simulink model "ZF02HD250606_23a"  (R2023a)
settings: Solver=ode4  StartTime=0.0  StopTime=inf  FixedStep=0.002  RelTol=1e-3
InitFcn:
  |  T_c = 0.002;
undefined symbols (not defined in the file): DiscIntNeverNeededParam, Discrete, magnitude, Time
libraries: AFCToolbox x33, simulink x28, simulink_extras x7, sharedtransform x2, ctrlSharedLib x2, aerolibconvert2 x1, aerolibtransform2 x1, dspstat3 x1, dspsolvers x1
(part 2 of 3)

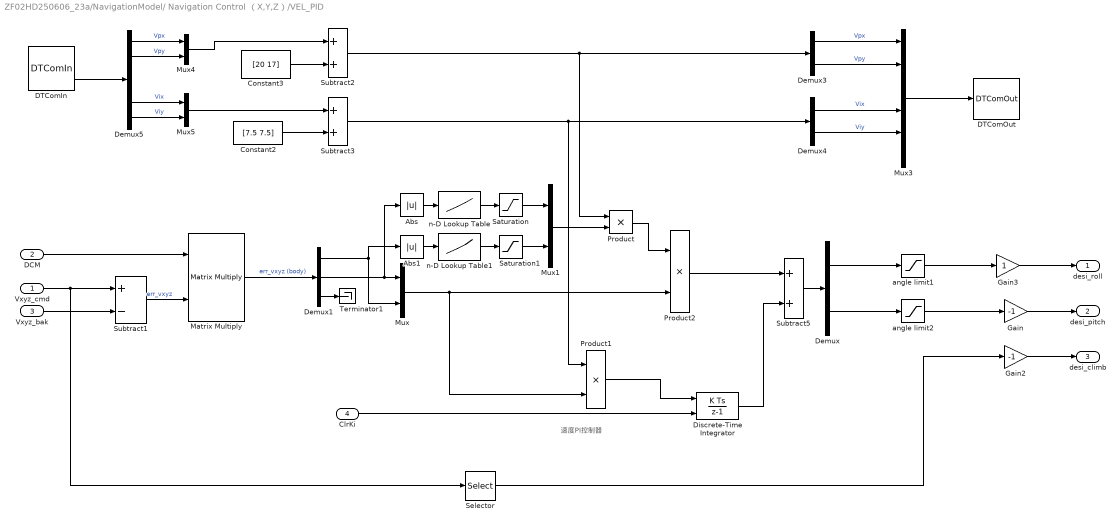
== system ZF02HD250606_23a/NavigationModel/ Navigation Control （X,Y,Z）/VEL_PID ==
  note: 速度PI控制器
  Vxyz_cmd : Inport
  DCM : Inport  Port=2
  Vxyz_bak : Inport  Port=3
  ClrKi : Inport  Port=4
  Abs : Abs  SaturateOnIntegerOverflow=off
  Abs1 : Abs  SaturateOnIntegerOverflow=off
  Constant2 : Constant  Value=[7.5 7.5]
  Constant3 : Constant  Value=[20 17]
  DTComIn : AFCToolbox/DeviceModule/DTComIn  Priority=2  g_sampleTime=0.01  g_frameType=21  g_resFrameNum=0  g_comPort=6  g_instName=0  g_id=0
      settings: SourceProductName=AFCToolbox
  DTComOut : AFCToolbox/DeviceModule/DTComOut  Priority=8  g_frameType=17  g_outFreq=50  g_comPort=0  g_instName=0  g_id=0
      settings: SourceProductName=AFCToolbox
  Demux : Demux  Outputs=2
  Demux1 : Demux  Outputs=3
  Demux3 : Demux  Outputs=2
  Demux4 : Demux  Outputs=2
  Demux5 : Demux  Outputs=6
  Discrete-Time Integrator : DiscreteIntegrator  ExternalReset=level  SampleTime=-1  LimitOutput=on  UpperSaturationLimit=5  LowerSaturationLimit=-5  ICPrevOutput=DiscIntNeverNeededParam  ICPrevScaledInput=DiscIntNeverNeededParam
  Gain : Gain  Gain=-1
  Gain2 : Gain  Gain=-1
  Gain3 : Gain
  Matrix Multiply : Product  Multiplication=Matrix(*)
  Mux{,1,4..5} (4 alike) : Mux  Inputs=2
  Mux3 : Mux  Inputs=6
  Product : Product
  Product1 : Product
  Product2 : Product
  Saturation : Saturate  UpperLimit=3  LowerLimit=1
  Saturation1 : Saturate  UpperLimit=3  LowerLimit=1
  Selector : Selector  InputPortWidth=3  IndexOptions=Index vector (dialog)  Indices=3  OutputSizes=1
  Subtract1 : Sum  Inputs=+-
  Subtract2 : Sum
  Subtract3 : Sum
  Subtract5 : Sum
  Terminator1 : Terminator
  angle limit1 : Saturate  UpperLimit=30  LowerLimit=-30
  angle limit2 : Saturate  UpperLimit=30  LowerLimit=-30
  n-D Lookup Table : Lookup_n-D  NumberOfTableDimensions=1  BreakpointsForDimension1=[0,0.4,5]  BreakpointsForDimension3=[5, 7]  Table=[2.5,1.5,1]  InternalRulePriority=Speed  RndMeth=Simplest
  n-D Lookup Table1 : Lookup_n-D  NumberOfTableDimensions=1  BreakpointsForDimension1=[0,0.4,5]  BreakpointsForDimension3=[5, 7]  Table=[3,1.5,1]  InternalRulePriority=Speed  RndMeth=Simplest
  desi_roll : Outport
  desi_pitch : Outport  Port=2
  desi_climb : Outport  Port=3
  wires:
  angle limit2/1 -> Gain/1
  angle limit1/1 -> Gain3/1
  Discrete-Time Integrator/1 -> Subtract5/2
  Demux/1 -> angle limit1/1
  Demux/2 -> angle limit2/1
  Gain/1 -> desi_pitch/1
  Gain3/1 -> desi_roll/1
  ClrKi/1 -> Discrete-Time Integrator/2
  Subtract5/1 -> Demux/1
  Gain2/1 -> desi_climb/1
  Selector/1 -> Gain2/1
  Demux1/1 -> Mux/2, Abs1/1
  Demux1/2 -> Abs/1, Mux/1
  Matrix Multiply/1 -> Demux1/1  "err_vxyz (body)"
  DCM/1 -> Matrix Multiply/1
  Vxyz_bak/1 -> Subtract1/2
  Subtract1/1 -> Matrix Multiply/2  "err_vxyz"
  Mux/1 -> Product1/2, Product2/2
  Demux3/2 -> Mux3/2  "Vpy"
  Demux3/1 -> Mux3/1  "Vpx"
  Demux4/1 -> Mux3/4  "Vix"
  Demux4/2 -> Mux3/5  "Viy"
  Mux3/1 -> DTComOut/1
  Product1/1 -> Discrete-Time Integrator/1
  Vxyz_cmd/1 -> Selector/1, Subtract1/1
  Demux1/3 -> Terminator1/1
  Subtract3/1 -> Product1/1, Demux4/1
  n-D Lookup Table1/1 -> Saturation1/1
  n-D Lookup Table/1 -> Saturation/1
  Product/1 -> Product2/1
  Product2/1 -> Subtract5/1
  Constant2/1 -> Subtract3/2
  Mux5/1 -> Subtract3/1
  Demux5/6 -> Mux5/2  "Viy"
  Demux5/5 -> Mux5/1  "Vix"
  Demux5/2 -> Mux4/2  "Vpy"
  Demux5/1 -> Mux4/1  "Vpx"
  DTComIn/2 -> Demux5/1
  Mux4/1 -> Subtract2/1
  Constant3/1 -> Subtract2/2
  Mux1/1 -> Product/2
  Subtract2/1 -> Product/1, Demux3/1
  Saturation/1 -> Mux1/1
  Saturation1/1 -> Mux1/2
  Abs/1 -> n-D Lookup Table/1
  Abs1/1 -> n-D Lookup Table1/1

== system ZF02HD250606_23a/NavigationModel/GPSNav/1 ==
  Cbn : Inport
  accl_ned_m/s2 : Inport  Port=2
  QGC_sensor_reinit : Inport  Port=3
  GPS_fixtype : Inport  Port=4
  GPS_V_m/s : Inport  Port=5
  GPS_LLA_rad : Inport  Port=6
  GPSHdop : Inport  Port=7
  Cast To Boolean : DataTypeConversion  OutDataTypeStr=double  SaturateOnIntegerOverflow=off  RndMeth=Floor
  Compare To Constant : simulink/Logic and Bit Operations/Compare To Constant  relop=>=  const=1  OutDataTypeStr=boolean
  Compare To Constant1 : simulink/Logic and Bit Operations/Compare To Constant  relop=>=  const=1  OutDataTypeStr=boolean
  GPS_Data_Process : Subsystem
  Logical Operator : Logic  AllPortsSameDT=off  OutDataTypeStr=boolean
  Translation_estimate : Subsystem
  vxy_estimout : Outport
  Pxy_estimout : Outport  Port=2
  posNE_gps : Outport  Port=3
  tag scope: AccelFusion_sta=global
  wires:
  Compare To Constant/1 -> Logical Operator/1
  GPS_Data_Process/1(init_GPSLLAflag) -> Compare To Constant1/1
  GPSHdop/1 -> Translation_estimate/6(GPSHdop), GPS_Data_Process/5(GPSHdop)
  QGC_sensor_reinit/1 -> Translation_estimate/7(QGC_init), GPS_Data_Process/4(QGC_sensor_reinit)
  GPS_LLA_rad/1 -> GPS_Data_Process/2(GPS_LLA_rad)
  GPS_V_m/s/1 -> GPS_Data_Process/1(GPS_V_m/s)
  accl_ned_m/s2/1 -> Translation_estimate/2(accl_ned_m/s2)
  Cbn/1 -> Translation_estimate/1(Cbn)
  GPS_Data_Process/2(vne_gps) -> Translation_estimate/3(vne_gps)
  GPS_Data_Process/3(posNE_gps) -> posNE_gps/1, Translation_estimate/4(posNE_gps1)
  GPS_fixtype/1 -> Compare To Constant/1, Translation_estimate/5(GPSstate), GPS_Data_Process/3(GPS_fixtype)  "sts"
  Translation_estimate/1(vxy_estimout) -> vxy_estimout/1
  Translation_estimate/2(Pxy_estimout) -> Pxy_estimout/1
  Cast To Boolean/1 -> [AccelFusion_sta]
  Compare To Constant1/1 -> Logical Operator/2
  Logical Operator/1 -> Translation_estimate/Enable, Cast To Boolean/1

== system ZF02HD250606_23a/BasicModel/AttiAltHold/ReturnShutOff/Subsystem ==
  In1 : Inport
  Add : Sum  Inputs=+-
  Constant : Constant  Value=iValue
  Constant1 : Constant  Value=0
  Switch1 : Switch  Criteria=u2 > Threshold  SaturateOnIntegerOverflow=off  InputSameDT=off
  Out1 : Outport
  wires:
  In1/1 -> Add/1
  Switch1/1 -> Out1/1
  Add/1 -> Switch1/2, Switch1/1
  Constant1/1 -> Switch1/3
  Constant/1 -> Add/2

== system ZF02HD250606_23a/BasicModel/AttiAltHold/Subsystem/If Action Subsystem ==
  iThrottle : Inport
  preThrottHover : Inport  Port=2
  Action Port : ActionPort  ActionPortLabel=if(u1 ~= 0)
  Add : Sum
  Gain : Gain  Gain=0.99
  Gain1 : Gain  Gain=0.01
  ThrottHover : Outport
  wires:
  preThrottHover/1 -> Gain/1
  iThrottle/1 -> Gain1/1
  Gain/1 -> Add/1
  Gain1/1 -> Add/2
  Add/1 -> ThrottHover/1

== system ZF02HD250606_23a/BasicModel/AttiAltHold/Subsystem/If Action Subsystem1 ==
  In1 : Inport
  Action Port : ActionPort  ActionPortLabel=else
  Out1 : Outport
  wires:
  In1/1 -> Out1/1

== system ZF02HD250606_23a/BasicModel/AttiAltHold/h_fusion1/judgement ==
  note: 输入为GPS的搜星数，搜星数>5时，GPS速度参与融合，flag置1；
      |                                              否则，GPS速度不参与融合，flag置0.
  starN : Inport
  If : If  IfExpression=u1 > 5
  If Action Subsystem : Subsystem  TreatAsAtomicUnit=on
  If Action Subsystem2 : Subsystem  TreatAsAtomicUnit=on
  Merge : Merge
  flag : Outport
  wires:
  If/1 -> If Action Subsystem/Action
  If Action Subsystem2/1(temp_value) -> Merge/2
  starN/1 -> If/1
  If Action Subsystem/1(temp_value) -> Merge/1
  Merge/1 -> flag/1
  If/2 -> If Action Subsystem2/Action

== system ZF02HD250606_23a/NavigationModel/ Navigation Control （X,Y,Z）/SETPOINT/Subsystem ==
  takeoff : Inport
  pos : Inport  Port=2
  Logical Operator : Logic  Operator=NOT  AllPortsSameDT=off  OutDataTypeStr=boolean
  Memory : Memory
  Switch : Switch  Criteria=u2 > Threshold  Threshold=0.5  SaturateOnIntegerOverflow=off  InputSameDT=off
  posxy : Outport
  wires:
  Switch/1 -> Memory/1, posxy/1
  Memory/1 -> Switch/3
  takeoff/1 -> Logical Operator/1
  pos/1 -> Switch/1
  Logical Operator/1 -> Switch/2

== system ZF02HD250606_23a/NavigationModel/ Navigation Control （X,Y,Z）/SETPOINT/return_mode1 ==
  pos1 : Inport
  posxy : Inport  Port=2  PortDimensions=[ 2 1]
  Enable : EnablePort
  Abs : Abs  SaturateOnIntegerOverflow=off
  Add1 : Sum  Inputs=+-
  Add4 : Sum  Inputs=+-
  Constant : Constant  Value=landing_pos
  Constant1 : Constant  Value=-decision_h
  Constant11 : Constant  Value=15
  Constant2 : Constant  Value=-decision_h
  Constant3 : Constant  Value=accept_radius_h
  Constant4 : Constant  Value=accept_radius
  Logical Operator : Logic  Operator=NOT  AllPortsSameDT=off  OutDataTypeStr=boolean
  Memory{1..4} (4 alike) : Memory
  Mux : Mux  Inputs=2
  Mux1 : Mux  Inputs=2
  Relational Operator1 : RelationalOperator  Operator=<=  OutDataTypeStr=boolean  RndMeth=Simplest  InputSameDT=off
  Relational Operator2 : RelationalOperator  Operator=<=  OutDataTypeStr=boolean  RndMeth=Simplest  InputSameDT=off
  Selector1 : Selector  InputPortWidth=3  IndexOptions=Index vector (dialog)  Indices=[3]  OutputSizes=1
  Selector6 : Selector  InputPortWidth=3  IndexOptions=Index vector (dialog)  Indices=[1 2]  OutputSizes=1
  Selector7 : Selector  InputPortWidth=3  IndexOptions=Index vector (dialog)  Indices=[1 2]  OutputSizes=1
  Switch{,1..2,4} (4 alike) : Switch  Criteria=u2 > Threshold  Threshold=0.5  SaturateOnIntegerOverflow=off  InputSameDT=off
  TD : Subsystem
  norm : Subsystem
  setpoint_next : Outport
  flag : Outport  Port=2
  wires:
  Add4/1 -> norm/1(u)
  Mux1/1 -> Switch1/1
  norm/1(y) -> Switch2/3
  Relational Operator1/1 -> Switch1/2, Memory1/1, Logical Operator/1
  Constant3/1 -> Relational Operator1/2
  posxy/1 -> Mux/1
  Relational Operator2/1 -> Memory3/1, Switch/2
  Selector6/1 -> Add4/1
  Constant2/1 -> Add1/2, Mux/2
  Constant4/1 -> Relational Operator2/2
  Memory1/1 -> Switch4/2
  Selector7/1 -> Add4/2, Mux1/1
  Memory3/1 -> Switch2/2
  Memory4/1 -> Switch2/1
  Mux/1 -> Switch1/3
  Switch2/1 -> Relational Operator2/1, Memory4/1
  Switch1/1 -> Switch/3
  Constant/1 -> Switch/1, Selector7/1
  Constant1/1 -> Mux1/2
  Memory2/1 -> Switch4/1
  Selector1/1 -> Add1/1
  Switch4/1 -> Relational Operator1/1, Memory2/1
  Add1/1 -> Abs/1
  Abs/1 -> Switch4/3
  Switch/1 -> TD/1(D)
  Constant11/1 -> TD/2(r)
  pos1/1 -> TD/3(r1), Selector1/1, Selector6/1
  TD/1(setpoint_next) -> setpoint_next/1
  Logical Operator/1 -> flag/1

== system ZF02HD250606_23a/NavigationModel/ Navigation Control （X,Y,Z）/SETPOINT/setpoints1 ==
  pos1 : Inport
  xyz_cmd : Inport  Port=2
  FLAG : Inport  Port=3
  Enable : EnablePort
  Add : Sum
  Add2 : Sum
  Chart : Stateflow chart  TreatAsAtomicUnit=on
  Constant1 : Constant
  Constant11 : Constant  Value=15
  Constant2 : Constant  Value=0
  Constant3 : Constant
  Constant4 : Constant  Value=accept_radius_1
  Constant5 : Constant  Value=setpoints
  Logical Operator : Logic  Operator=OR  AllPortsSameDT=off  OutDataTypeStr=boolean
  Memory : Memory  InheritSampleTime=on
  Relational Operator2 : RelationalOperator  Operator=<=  OutDataTypeStr=boolean  RndMeth=Simplest  InputSameDT=off
  Saturation : Saturate  UpperLimit=size(setpoints,1)  LowerLimit=1
  Selector1 : Selector  NumberOfDimensions=2  InputPortWidth=4  IndexOptions=Index vector (port),Select all  Indices=[1 3],1  OutputSizes=1,1
  Subtract : Sum  Inputs=+-
  Switch : Switch  Criteria=u2 > Threshold  SaturateOnIntegerOverflow=off  InputSameDT=off
  Switch5 : Switch  Criteria=u2 > Threshold  Threshold=0.5  SaturateOnIntegerOverflow=off  InputSameDT=off
  TD : Subsystem
  Transpose1 : Math  Operator=transpose  SignedPower=on
  norm : Subsystem
  setpoint_next : Outport
  Flag : Outport  Port=2
  wires:
  Relational Operator2/1 -> Chart/1(dist)
  norm/1(y) -> Relational Operator2/1
  Selector1/1 -> Transpose1/1
  Constant3/1 -> Add2/2
  Add/1 -> Memory/1
  Saturation/1 -> Selector1/2
  Constant4/1 -> Relational Operator2/2
  Constant1/1 -> Switch/1
  Memory/1 -> Add/2, Add2/1
  Constant2/1 -> Switch/3
  Switch/1 -> Add/1
  Add2/1 -> Saturation/1
  Subtract/1 -> norm/1(u)
  Chart/1(flag_setpoint) -> Logical Operator/1, Switch/2
  Constant5/1 -> Selector1/1
  xyz_cmd/1 -> Switch5/1
  FLAG/1 -> Logical Operator/2, Switch5/2
  Transpose1/1 -> Subtract/2, Switch5/3
  pos1/1 -> Subtract/1, TD/3(r1)
  Constant11/1 -> TD/2(r)
  Switch5/1 -> TD/1(D)
  TD/1(setpoint_next) -> setpoint_next/1
  Logical Operator/1 -> Flag/1

== system ZF02HD250606_23a/NavigationModel/ Navigation Control （X,Y,Z）/SETPOINT/takeoff2 ==
  posxy : Inport
  h : Inport  Port=2
  Enable : EnablePort
  Abs : Abs  SaturateOnIntegerOverflow=off
  Add : Sum  Inputs=+-
  Compare To Constant1 : simulink/Logic and Bit Operations/Compare To Constant  relop=<=  const=0.3  OutDataTypeStr=boolean
  Constant : Constant  Value=takeoff_h
  Constant5 : Constant  Value=setpoint1
  Memory : Memory
  Memory3 : Memory
  Mux : Mux  Inputs=2
  Mux1 : Mux  Inputs=2
  Switch : Switch  Criteria=u2 > Threshold  Threshold=0.5  SaturateOnIntegerOverflow=off  InputSameDT=off
  Switch1 : Switch  Criteria=u2 > Threshold  Threshold=0.5  SaturateOnIntegerOverflow=off  InputSameDT=off
  setpoint_next : Outport
  flag : Outport  Port=2
  wires:
  Constant5/1 -> Mux/1
  Constant/1 -> Add/1, Mux1/2, Mux/2
  posxy/1 -> Mux1/1
  h/1 -> Add/2
  Add/1 -> Abs/1
  Abs/1 -> Switch1/3
  Mux/1 -> Switch/1
  Mux1/1 -> Switch/3
  Memory/1 -> Switch1/1
  Switch1/1 -> Memory/1, Compare To Constant1/1
  Compare To Constant1/1 -> Switch/2, flag/1, Memory3/1
  Memory3/1 -> Switch1/2
  Switch/1 -> setpoint_next/1

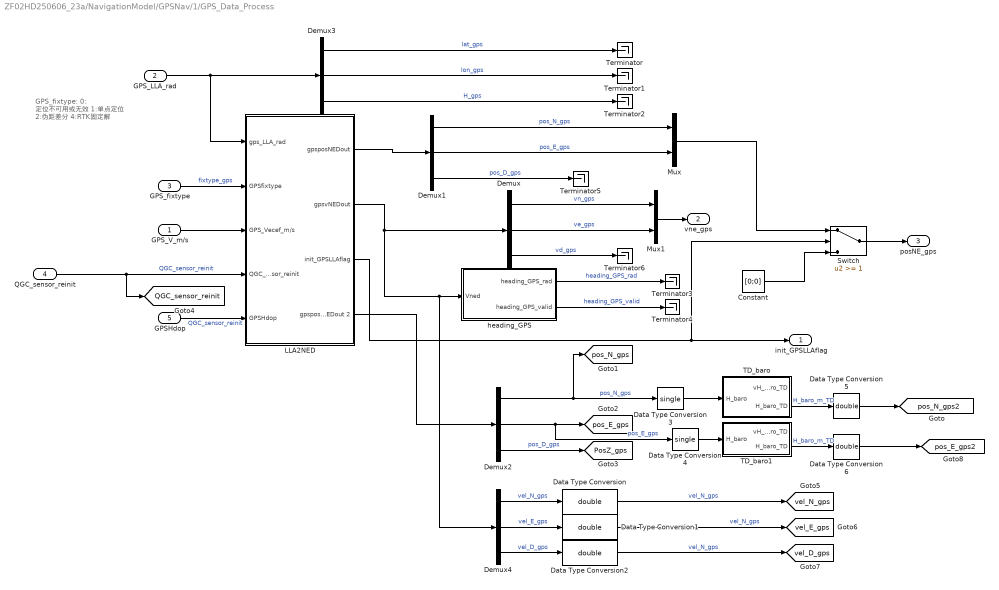
== system ZF02HD250606_23a/NavigationModel/GPSNav/1/GPS_Data_Process ==
  note: GPS_fixtype:
      | 0: 定位不可用或无效
      | 1:单点定位
      | 2:伪距差分
      | 4:RTK固定解
  GPS_V_m/s : Inport
  GPS_LLA_rad : Inport  Port=2
  GPS_fixtype : Inport  Port=3
  QGC_sensor_reinit : Inport  Port=4
  GPSHdop : Inport  Port=5
  Constant : Constant  Value=[0;0]
  Data Type Conversion{,1..2,5..6} (5 alike) : DataTypeConversion  OutDataTypeStr=double  SaturateOnIntegerOverflow=off  RndMeth=Floor
  Data Type Conversion3 : DataTypeConversion  OutDataTypeStr=single  SaturateOnIntegerOverflow=off  RndMeth=Floor
  Data Type Conversion4 : DataTypeConversion  OutDataTypeStr=single  SaturateOnIntegerOverflow=off  RndMeth=Floor
  Demux{,1..4} (5 alike) : Demux  Outputs=3
  LLA2NED : Subsystem
  Mux : Mux  Inputs=2
  Mux1 : Mux  Inputs=2
  Switch : Switch  Threshold=1  SaturateOnIntegerOverflow=off  InputSameDT=off
  TD_baro : Subsystem
  TD_baro1 : Subsystem
  Terminator{,1..6} (7 alike) : Terminator
  heading_GPS : Subsystem
  init_GPSLLAflag : Outport
  vne_gps : Outport  Port=2
  posNE_gps : Outport  Port=3
  tag scope: PosZ_gps=global, QGC_sensor_reinit=global, pos_E_gps2=global, pos_E_gps=global, pos_N_gps2=global, pos_N_gps=global, vel_D_gps=global, vel_E_gps=global, vel_N_gps=global
  wires:
  GPS_fixtype/1 -> LLA2NED/2(GPSfixtype)  "fixtype_gps"
  Demux3/3 -> Terminator2/1  "H_gps"
  Demux/3 -> Terminator6/1  "vd_gps"
  Demux/1 -> Mux1/1  "vn_gps"
  GPS_LLA_rad/1 -> Demux3/1, LLA2NED/1(gps_LLA_rad)
  Demux/2 -> Mux1/2  "ve_gps"
  Demux3/2 -> Terminator1/1  "lon_gps"
  Demux3/1 -> Terminator/1  "lat_gps"
  QGC_sensor_reinit/1 -> [QGC_sensor_reinit], LLA2NED/4(QGC_sensor_reinit)  "QGC_sensor_reinit"
  LLA2NED/1("gpsposNEDout ") -> Demux1/1
  Demux1/1 -> Mux/1  "pos_N_gps"
  Demux1/2 -> Mux/2  "pos_E_gps"
  Demux1/3 -> Terminator5/1  "pos_D_gps"
  GPS_V_m/s/1 -> LLA2NED/3(GPS_Vecef_m/s)
  LLA2NED/2(gpsvNEDout) -> Demux4/1, heading_GPS/1(Vned), Demux/1
  heading_GPS/1(heading_GPS_rad) -> Terminator3/1  "heading_GPS_rad"
  heading_GPS/2(heading_GPS_valid) -> Terminator4/1  "heading_GPS_valid"
  Mux/1 -> Switch/1
  Mux1/1 -> vne_gps/1
  GPSHdop/1 -> LLA2NED/5(GPSHdop)  "QGC_sensor_reinit"
  LLA2NED/3(init_GPSLLAflag) -> Switch/2, init_GPSLLAflag/1
  Constant/1 -> Switch/3
  Switch/1 -> posNE_gps/1
  Demux2/1 -> [pos_N_gps], Data Type Conversion3/1  "pos_N_gps"
  Demux2/3 -> [PosZ_gps]  "pos_D_gps"
  Demux2/2 -> Data Type Conversion4/1, [pos_E_gps]  "pos_E_gps"
  LLA2NED/4(gpsposNEDout 2) -> Demux2/1
  Demux4/2 -> Data Type Conversion1/1  "vel_E_gps"
  Demux4/3 -> Data Type Conversion2/1  "vel_D_gps"
  Demux4/1 -> Data Type Conversion/1  "vel_N_gps"
  Data Type Conversion/1 -> [vel_N_gps]  "vel_N_gps"
  Data Type Conversion1/1 -> [vel_E_gps]  "vel_N_gps"
  Data Type Conversion2/1 -> [vel_D_gps]  "vel_N_gps"
  TD_baro/2(H_baro_TD) -> Data Type Conversion5/1  "H_baro_m_TD"
  TD_baro1/2(H_baro_TD) -> Data Type Conversion6/1  "H_baro_m_TD"
  Data Type Conversion3/1 -> TD_baro/1(H_baro)
  Data Type Conversion4/1 -> TD_baro1/1(H_baro)
  Data Type Conversion5/1 -> [pos_N_gps2]
  Data Type Conversion6/1 -> [pos_E_gps2]

== system ZF02HD250606_23a/NavigationModel/GPSNav/1/Translation_estimate ==
  Cbn : Inport
  accl_ned_m/s2 : Inport  Port=2
  vne_gps : Inport  Port=3
  posNE_gps1 : Inport  Port=4
  GPSstate : Inport  Port=5
  GPSHdop : Inport  Port=6
  QGC_init : Inport  Port=7
  Enable : EnablePort
  Subsystem : Subsystem
  Subsystem2 : Subsystem
  V_Horizontal_estimation1 : Subsystem  Commented=on
  translate to N : Subsystem
  vxy_estimout : Outport
  Pxy_estimout : Outport  Port=2
  wires:
  Cbn/1 -> translate to N/1(Cbn)
  accl_ned_m/s2/1 -> translate to N/2(accl_ned)
  QGC_init/1 -> Subsystem/4(QGC_init), Subsystem2/3(QGC_init)
  posNE_gps1/1 -> Subsystem/2(pxy_GPS)
  GPSHdop/1 -> Subsystem2/4(DOP), Subsystem/5(DOP)
  Subsystem/1(pxy_est) -> Pxy_estimout/1
  Subsystem2/1(vxy_est) -> vxy_estimout/1, Subsystem/1(vxy)
  translate to N/1(accel_Horizontal_predict) -> Subsystem2/1(axy)
  vne_gps/1 -> Subsystem2/2(vxy_GPS)
  Subsystem2/2(GPSv_enable) -> Subsystem/3(GPSv_enable)

== system ZF02HD250606_23a/BasicModel/AttiAltHold/h_fusion1/judgement/If Action Subsystem ==
  Action Port : ActionPort  ActionPortLabel=if(u1 > 5)
  Constant : Constant
  temp_value : Outport
  wires:
  Constant/1 -> temp_value/1

== system ZF02HD250606_23a/BasicModel/AttiAltHold/h_fusion1/judgement/If Action Subsystem2 ==
  Action Port : ActionPort  ActionPortLabel=else
  Constant : Constant  Value=0
  temp_value : Outport
  wires:
  Constant/1 -> temp_value/1

== system ZF02HD250606_23a/NavigationModel/ Navigation Control （X,Y,Z）/SETPOINT/return_mode1/TD ==
  D : Inport
  r : Inport  Port=2
  r1 : Inport  Port=3
  Constant1 : Constant  Value=0.01
  Discrete-Time Integrator1 : DiscreteIntegrator  InitialConditionSource=external  SampleTime=-1  ICPrevOutput=DiscIntNeverNeededParam  ICPrevScaledInput=DiscIntNeverNeededParam
  Discrete-Time Integrator3 : DiscreteIntegrator  SampleTime=-1  ICPrevOutput=DiscIntNeverNeededParam  ICPrevScaledInput=DiscIntNeverNeededParam
  Fhan : Subsystem
  Sum24 : Sum  Inputs=|-+
  x1 : Scope
  x2 : Scope
  setpoint_next : Outport
  wires:
  Fhan/1(fh) -> Discrete-Time Integrator3/1
  Constant1/1 -> Fhan/4(h)
  Discrete-Time Integrator1/1 -> setpoint_next/1, Sum24/2, x1/1  "x1"
  D/1 -> Sum24/1
  Sum24/1 -> Fhan/1(x1)
  Discrete-Time Integrator3/1 -> x2/1, Discrete-Time Integrator1/1, Fhan/2(x2)  "x2"
  r/1 -> Fhan/3(r)
  r1/1 -> Discrete-Time Integrator1/2

== system ZF02HD250606_23a/NavigationModel/ Navigation Control （X,Y,Z）/SETPOINT/return_mode1/norm ==
  u : Inport
  Product : Product
  Sqrt : Sqrt
  Sum of Elements : Sum  Inputs=+
  y : Outport
  wires:
  Sum of Elements/1 -> Sqrt/1
  Product/1 -> Sum of Elements/1
  u/1 -> Product/2, Product/1
  Sqrt/1 -> y/1

== system ZF02HD250606_23a/NavigationModel/ Navigation Control （X,Y,Z）/SETPOINT/setpoints1/TD ==
  D : Inport
  r : Inport  Port=2
  r1 : Inport  Port=3
  Constant1 : Constant  Value=0.01
  Discrete-Time Integrator1 : DiscreteIntegrator  InitialConditionSource=external  SampleTime=-1  ICPrevOutput=DiscIntNeverNeededParam  ICPrevScaledInput=DiscIntNeverNeededParam
  Discrete-Time Integrator3 : DiscreteIntegrator  SampleTime=-1  ICPrevOutput=DiscIntNeverNeededParam  ICPrevScaledInput=DiscIntNeverNeededParam
  Fhan : Subsystem
  Sum24 : Sum  Inputs=|-+
  x1 : Scope
  x2 : Scope
  setpoint_next : Outport
  wires:
  Fhan/1(fh) -> Discrete-Time Integrator3/1
  Constant1/1 -> Fhan/4(h)
  Discrete-Time Integrator1/1 -> setpoint_next/1, Sum24/2, x1/1  "x1"
  D/1 -> Sum24/1
  Sum24/1 -> Fhan/1(x1)
  Discrete-Time Integrator3/1 -> x2/1, Discrete-Time Integrator1/1, Fhan/2(x2)  "x2"
  r/1 -> Fhan/3(r)
  r1/1 -> Discrete-Time Integrator1/2

== system ZF02HD250606_23a/NavigationModel/ Navigation Control （X,Y,Z）/SETPOINT/setpoints1/norm ==
  u : Inport
  Product : Product
  Sqrt : Sqrt
  Sum of Elements : Sum  Inputs=+
  y : Outport
  wires:
  Sum of Elements/1 -> Sqrt/1
  Product/1 -> Sum of Elements/1
  u/1 -> Product/2, Product/1
  Sqrt/1 -> y/1

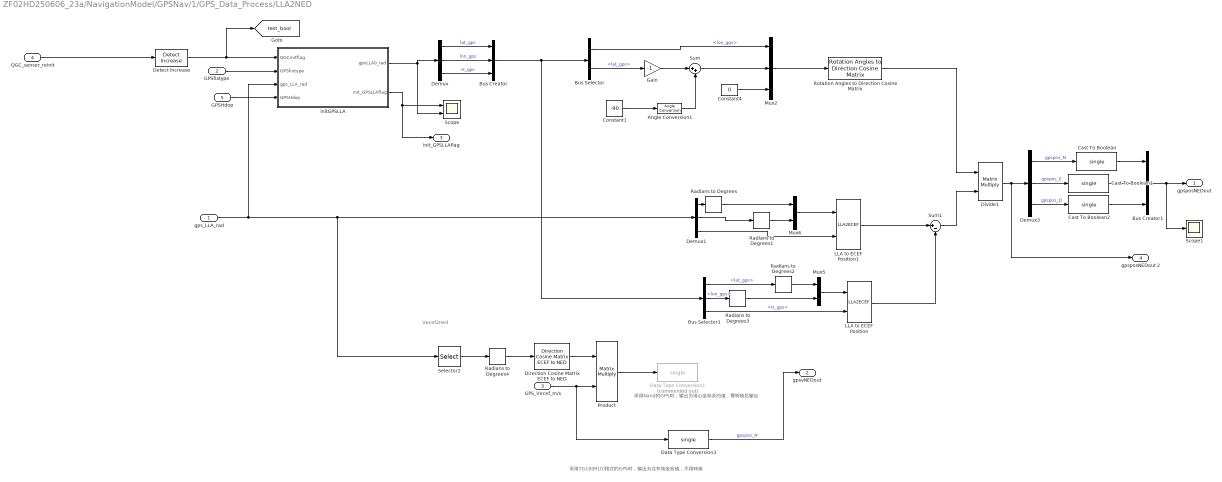
== system ZF02HD250606_23a/NavigationModel/GPSNav/1/GPS_Data_Process/LLA2NED ==
  note: 采用TG18(M10)格式的GPS时，输出为北东地坐标值，不用转换
  note: Vecef2ned
  note: 采用Nand的GPS时，输出为地心坐标系的值，需转换后输出
  gps_LLA_rad : Inport
  GPSfixtype : Inport  Port=2
  GPS_Vecef_m/s : Inport  Port=3
  QGC_sensor_reinit : Inport  Port=4
  GPSHdop : Inport  Port=5
  Angle Conversion1 : aerolibconvert2/Angle Conversion  IU=deg  OU=rad
  Bus Creator : BusCreator  Inputs=3
  Bus Creator1 : BusCreator  Inputs=3
  Bus Selector : BusSelector  OutputSignals=lon_gps,lat_gps
  Bus Selector1 : BusSelector  OutputSignals=lat_gps,lon_gps,H_gps
  Cast To Boolean : DataTypeConversion  OutDataTypeStr=single  SaturateOnIntegerOverflow=off  RndMeth=Floor
  Cast To Boolean1 : DataTypeConversion  OutDataTypeStr=single  SaturateOnIntegerOverflow=off  RndMeth=Floor
  Cast To Boolean2 : DataTypeConversion  OutDataTypeStr=single  SaturateOnIntegerOverflow=off  RndMeth=Floor
  Constant1 : Constant  Value=-90
  Constant4 : Constant  Value=0
  Data Type Conversion1 : DataTypeConversion  Commented=on  OutDataTypeStr=single  SaturateOnIntegerOverflow=off  RndMeth=Floor
  Data Type Conversion3 : DataTypeConversion  OutDataTypeStr=single  SaturateOnIntegerOverflow=off  RndMeth=Floor
  Demux : Demux  Outputs=3
  Demux1 : Demux  Outputs=3
  Demux3 : Demux  Outputs=3
  Detect Increase : simulink/Logic and Bit Operations/Detect Increase  vinit=0.0  OutDataTypeStr=boolean
  Direction Cosine Matrix ECEF to NED : aerolibtransform2/Direction Cosine Matrix ECEF to NED
  Divide1 : Product  Inputs=**  Multiplication=Matrix(*)
  Gain : Gain  Gain=-1
  LLA to ECEF Position : LLA2ECEF  R=6378137
  LLA to ECEF Position1 : LLA2ECEF  R=6378137
  Mux2 : Mux  Inputs=3
  Mux5 : Mux  Inputs=2
  Mux6 : Mux  Inputs=2
  Product : Product  Multiplication=Matrix(*)
  Radians to Degrees{,1..4} (5 alike) : simulink_extras/Transformations/Radians to Degrees
  Rotation Angles to Direction Cosine Matrix : sharedtransform/Rotation Angles to Direction Cosine Matrix  rotationOrder=ZYX  aMode=aMode
  Scope : Scope  NumInputPorts=2
  Scope1 : Scope
  Selector2 : Selector  InputPortWidth=3  IndexOptions=Index vector (dialog)  Indices=[1 2]  OutputSizes=1
  Sum : Sum  Inputs=|++
  Sum1 : Sum  Inputs=|+-
  initGPSLLA : MATLAB Function  TreatAsAtomicUnit=on
  "gpsposNEDout " : Outport
  gpsvNEDout : Outport  Port=2
  init_GPSLLAflag : Outport  Port=3
  gpsposNEDout 2 : Outport  Port=4
  tag scope: test_bool=global
  wires:
  GPSfixtype/1 -> initGPSLLA/2(GPSfixtype)
  Bus Creator1/1 -> Scope1/1, "gpsposNEDout "/1
  Demux3/3 -> Cast To Boolean2/1  "gpspos_D"
  Demux3/2 -> Cast To Boolean1/1  "gpspos_E"
  Demux3/1 -> Cast To Boolean/1  "gpspos_N"
  Bus Creator/1 -> Bus Selector/1, Bus Selector1/1
  Demux/3 -> Bus Creator/3  "H_gps"
  Demux/2 -> Bus Creator/2  "lon_gps"
  Demux/1 -> Bus Creator/1  "lat_gps"
  Demux1/3 -> LLA to ECEF Position1/2
  Mux6/1 -> LLA to ECEF Position1/1
  Mux5/1 -> LLA to ECEF Position/1
  Gain/1 -> Sum/1
  LLA to ECEF Position1/1 -> Sum1/1
  Constant4/1 -> Mux2/3
  Sum1/1 -> Divide1/2
  Divide1/1 -> gpsposNEDout 2/1, Demux3/1
  Demux1/1 -> Radians to Degrees/1
  Mux2/1 -> Rotation Angles to Direction Cosine Matrix/1
  Rotation Angles to Direction Cosine Matrix/1 -> Divide1/1
  Constant1/1 -> Angle Conversion1/1
  LLA to ECEF Position/1 -> Sum1/2
  Demux1/2 -> Radians to Degrees1/1
  Sum/1 -> Mux2/2
  Bus Selector/2 -> Gain/1  "<lat_gps>"
  Bus Selector/1 -> Mux2/1  "<lon_gps>"
  Bus Selector1/1 -> Radians to Degrees2/1  "<lat_gps>"
  Bus Selector1/2 -> Radians to Degrees3/1  "<lon_gps>"
  Bus Selector1/3 -> LLA to ECEF Position/2  "<H_gps>"
  gps_LLA_rad/1 -> initGPSLLA/3(gps_LLA_rad), Selector2/1, Demux1/1
  Radians to Degrees/1 -> Mux6/1
  Radians to Degrees1/1 -> Mux6/2
  Angle Conversion1/1 -> Sum/2
  Radians to Degrees2/1 -> Mux5/1
  Radians to Degrees3/1 -> Mux5/2
  Direction Cosine Matrix ECEF to NED/1 -> Product/1
  Selector2/1 -> Radians to Degrees4/1
  Radians to Degrees4/1 -> Direction Cosine Matrix ECEF to NED/1
  Data Type Conversion3/1 -> gpsvNEDout/1  "gpspos_N"
  Detect Increase/1 -> [test_bool], initGPSLLA/1(QGCinitflag)
  initGPSLLA/1(gpsLLA0_rad) -> Demux/1, Scope/2
  initGPSLLA/2(init_GPSLLAflag) -> init_GPSLLAflag/1, Scope/1
  GPSHdop/1 -> initGPSLLA/4(GPSHdop)
  Cast To Boolean/1 -> Bus Creator1/1
  Cast To Boolean1/1 -> Bus Creator1/2
  Cast To Boolean2/1 -> Bus Creator1/3
  QGC_sensor_reinit/1 -> Detect Increase/1
  GPS_Vecef_m/s/1 -> Data Type Conversion3/1, Product/2
  Product/1 -> Data Type Conversion1/1

== system ZF02HD250606_23a/NavigationModel/GPSNav/1/GPS_Data_Process/TD_baro ==
  H_baro : Inport
  Constant1 : Constant  Value=0.002  OutDataTypeStr=double
  Constant3 : Constant  Value=0.23  OutDataTypeStr=double
  Constant4 : Constant  Value=900  OutDataTypeStr=single
  Data Type Conversion : DataTypeConversion  OutDataTypeStr=single  SaturateOnIntegerOverflow=off  RndMeth=Floor
  Data Type Conversion1 : DataTypeConversion  OutDataTypeStr=single  SaturateOnIntegerOverflow=off  RndMeth=Floor
  Data Type Conversion5 : DataTypeConversion  OutDataTypeStr=single  SaturateOnIntegerOverflow=off  RndMeth=Floor
  Delay1 : Delay  DelayLength=1  InitialConditionSource=Input port
      settings: InputPortMap=u0,p4
  MATLAB Function2 : MATLAB Function  TreatAsAtomicUnit=on
  Memory : Memory  InheritSampleTime=on
  Scope : Scope  NumInputPorts=3
  vH_baro_TD : Outport
  H_baro_TD : Outport  Port=2
  wires:
  Delay1/1 -> H_baro_TD/1, Scope/3, MATLAB Function2/3("u1 ")
  H_baro/1 -> Data Type Conversion5/1
  Memory/1 -> MATLAB Function2/4("u2 "), vH_baro_TD/1, Scope/2
  Constant3/1 -> Data Type Conversion1/1
  Constant4/1 -> MATLAB Function2/6(r)
  MATLAB Function2/1(u1) -> Delay1/1
  MATLAB Function2/2(u2) -> Memory/1
  Data Type Conversion5/1 -> Scope/1, Delay1/2, MATLAB Function2/2(u0)
  Constant1/1 -> Data Type Conversion/1
  Data Type Conversion/1 -> MATLAB Function2/1(T)
  Data Type Conversion1/1 -> MATLAB Function2/5(h)

== system ZF02HD250606_23a/NavigationModel/GPSNav/1/GPS_Data_Process/TD_baro1 ==
  H_baro : Inport
  Constant1 : Constant  Value=0.002  OutDataTypeStr=double
  Constant3 : Constant  Value=0.23  OutDataTypeStr=double
  Constant4 : Constant  Value=900  OutDataTypeStr=single
  Data Type Conversion : DataTypeConversion  OutDataTypeStr=single  SaturateOnIntegerOverflow=off  RndMeth=Floor
  Data Type Conversion1 : DataTypeConversion  OutDataTypeStr=single  SaturateOnIntegerOverflow=off  RndMeth=Floor
  Data Type Conversion5 : DataTypeConversion  OutDataTypeStr=single  SaturateOnIntegerOverflow=off  RndMeth=Floor
  Delay1 : Delay  DelayLength=1  InitialConditionSource=Input port
      settings: InputPortMap=u0,p4
  MATLAB Function2 : MATLAB Function  TreatAsAtomicUnit=on
  Memory : Memory  InheritSampleTime=on
  Scope : Scope  NumInputPorts=3
  vH_baro_TD : Outport
  H_baro_TD : Outport  Port=2
  wires:
  Data Type Conversion5/1 -> MATLAB Function2/2(u0), Delay1/2, Scope/1
  MATLAB Function2/2(u2) -> Memory/1
  MATLAB Function2/1(u1) -> Delay1/1
  Constant4/1 -> MATLAB Function2/6(r)
  Constant1/1 -> Data Type Conversion/1
  Constant3/1 -> Data Type Conversion1/1
  Memory/1 -> Scope/2, vH_baro_TD/1, MATLAB Function2/4("u2 ")
  H_baro/1 -> Data Type Conversion5/1
  Delay1/1 -> MATLAB Function2/3("u1 "), Scope/3, H_baro_TD/1
  Data Type Conversion/1 -> MATLAB Function2/1(T)
  Data Type Conversion1/1 -> MATLAB Function2/5(h)

== system ZF02HD250606_23a/NavigationModel/GPSNav/1/GPS_Data_Process/heading_GPS ==
  Vned : Inport
  Atan2 : Trigonometry  Operator=atan2
  Compare To Constant : simulink/Logic and Bit Operations/Compare To Constant  relop=>  const=0.8  OutDataTypeStr=boolean
  Data Type Conversion : DataTypeConversion  OutDataTypeStr=double  SaturateOnIntegerOverflow=off  RndMeth=Floor
  Math Function : Math  Operator=magnitude^2  SignedPower=on
  Moving Average1 : dspstat3/Moving Average  Commented=on  Method=Sliding window  ForgettingFactorPort=off  SpecifyWindowLength=on  WindowLength=10  OverlapLength=9  AllowArbitraryInputLength=off  ForgettingFactor=0.9  SimulateUsing=Code generation
  Rate Transition : RateTransition  OutPortSampleTime=1
  Scope : Scope  NumInputPorts=2
  Scope1 : Scope
  Selector2 : Selector  InputPortWidth=3  IndexOptions=Index vector (dialog)  Indices=[2]  OutputSizes=1
  Selector3 : Selector  InputPortWidth=3  IndexOptions=Index vector (dialog)  Indices=[1]  OutputSizes=1
  Selector4 : Selector  InputPortWidth=3  IndexOptions=Index vector (dialog)  Indices=[1 2]  OutputSizes=1
  Sqrt : Sqrt
  Sum of Elements : Sum  Inputs=+
  heading_GPS_rad : Outport
  heading_GPS_valid : Outport  Port=2
  wires:
  Selector2/1 -> Atan2/1
  Math Function/1 -> Sum of Elements/1
  Vned/1 -> Selector2/1, Selector4/1, Selector3/1
  Selector3/1 -> Atan2/2
  Sum of Elements/1 -> Sqrt/1
  Selector4/1 -> Math Function/1
  Sqrt/1 -> Data Type Conversion/1
  Compare To Constant/1 -> Scope1/1, heading_GPS_valid/1
  Rate Transition/1 -> Scope/1, Scope/2, heading_GPS_rad/1
  Atan2/1 -> Rate Transition/1
  Data Type Conversion/1 -> Compare To Constant/1

== system ZF02HD250606_23a/NavigationModel/GPSNav/1/Translation_estimate/Subsystem ==
  vxy : Inport
  pxy_GPS : Inport  Port=2
  GPSv_enable : Inport  Port=3
  QGC_init : Inport  Port=4
  DOP : Inport  Port=5
  Add : Sum  Inputs=+-
  Add1 : Sum  Inputs=++-
  Compare To Constant : simulink/Logic and Bit Operations/Compare To Constant  relop=<=  const=3  OutDataTypeStr=boolean
  Delay : Delay  DelayLength=1  InitialCondition=[0;0;]  ExternalReset=Rising
      settings: InputPortMap=u0,r5
  Detect Change : simulink/Logic and Bit Operations/Detect Change  vinit=0  OutDataTypeStr=boolean
  Gain : Gain  Gain=0.002
  Kalman Filter : ctrlSharedLib/Kalman Filter  TimeDomain=Discrete-Time  UseCurrentEstimator=on  ModelSource=Individual A, B, C, D matrices  ModelSourceVariable=ss(0.95,1,1,0,1)  A=[0.1,0;0,0.1]  B=eye(2)  C=eye(2)  D=0  NumberOfStates=1  NumberOfInputs=1  NumberOfOutputs=1  InitialEstimateSource=Dialog  X0=0  P0=10  UseK=off  UseGH=off  NumberOfProcessNoiseInputs=1  G=1  TimeInvariantG=on  H=0  TimeInvariantH=on  Q=diag([0.1;0.1])  TimeInvariantQ=on  R=diag([0.8;0.8])  TimeInvariantR=on  N=0  TimeInvariantN=on  AddInputPort=off  AddEnablePort=on  ExternalReset=Rising  OutputEstimatedY=off  OutputP=off  Ts=-1
  Logical Operator : Logic  AllPortsSameDT=off  OutDataTypeStr=boolean
  Memory : Memory
  Product : Product  OutDataTypeStr=double
  QGC_init1 : InportShadow  Port=4
  Rate Transition1 : RateTransition  OutPortSampleTime=0.002
  Rate Transition2 : RateTransition  OutPortSampleTime=0.002
  Rate Transition3 : RateTransition  OutPortSampleTime=0.002
  Scope7 : Scope
  Selector : Selector  InputPortWidth=2  IndexOptions=Index vector (dialog)  Indices=[1]  OutputSizes=1
  pxy_est : Outport
  wires:
  Gain/1 -> Add1/1
  Delay/1 -> Add1/2
  Kalman Filter/1 -> Product/1
  pxy_GPS/1 -> Selector/1, Add/2
  Selector/1 -> Detect Change/1
  Product/1 -> Memory/1
  Logical Operator/1 -> Product/2, Rate Transition2/1
  Rate Transition2/1 -> Scope7/1, Kalman Filter/2
  Rate Transition1/1 -> Kalman Filter/1
  Memory/1 -> Add1/3
  Add/1 -> Rate Transition1/1
  vxy/1 -> Gain/1
  Add1/1 -> Add/1, Delay/1, pxy_est/1
  QGC_init/1 -> Rate Transition3/1
  Rate Transition3/1 -> Kalman Filter/3
  DOP/1 -> Compare To Constant/1
  Compare To Constant/1 -> Logical Operator/2
  QGC_init1/1 -> Delay/2
  GPSv_enable/1 -> Logical Operator/1

== system ZF02HD250606_23a/NavigationModel/GPSNav/1/Translation_estimate/Subsystem2 ==
  axy : Inport
  vxy_GPS : Inport  Port=2
  QGC_init : Inport  Port=3
  DOP : Inport  Port=4
  Add : Sum  Inputs=+-
  Add1 : Sum  Inputs=++-
  Compare To Constant : simulink/Logic and Bit Operations/Compare To Constant  relop=<=  const=3  OutDataTypeStr=boolean
  Delay : Delay  DelayLength=1  ExternalReset=Rising
      settings: InputPortMap=u0,r5
  Detect Change : simulink/Logic and Bit Operations/Detect Change  vinit=0  OutDataTypeStr=boolean
  Gain : Gain  Gain=0.002
  Kalman Filter : ctrlSharedLib/Kalman Filter  TimeDomain=Discrete-Time  UseCurrentEstimator=on  ModelSource=Individual A, B, C, D matrices  ModelSourceVariable=ss(0.95,1,1,0,1)  A=[0.6,0;0,0.6]  B=eye(2)  C=eye(2)  D=0  NumberOfStates=1  NumberOfInputs=1  NumberOfOutputs=1  InitialEstimateSource=Dialog  X0=0  P0=10  UseK=off  UseGH=off  NumberOfProcessNoiseInputs=1  G=1  TimeInvariantG=on  H=0  TimeInvariantH=on  Q=diag([0.1;0.1])  TimeInvariantQ=on  R=diag([0.6;0.6])  TimeInvariantR=on  N=0  TimeInvariantN=on  AddInputPort=off  AddEnablePort=on  ExternalReset=Rising  OutputEstimatedY=off  OutputP=off  Ts=-1
  Logical Operator : Logic  AllPortsSameDT=off  OutDataTypeStr=boolean
  Memory : Memory
  Product : Product  OutDataTypeStr=double
  Rate Transition1 : RateTransition  OutPortSampleTime=0.002
  Rate Transition2 : RateTransition  OutPortSampleTime=0.002
  Rate Transition3 : RateTransition  OutPortSampleTime=0.002
  Scope : Scope  NumInputPorts=2
  Scope7 : Scope
  Selector : Selector  InputPortWidth=2  IndexOptions=Index vector (dialog)  Indices=[1]  OutputSizes=1
  vxy_est : Outport
  GPSv_enable : Outport  Port=2
  wires:
  Compare To Constant/1 -> Logical Operator/2
  DOP/1 -> Compare To Constant/1
  Detect Change/1 -> Logical Operator/1
  Rate Transition3/1 -> Kalman Filter/3
  QGC_init/1 -> Delay/2, Rate Transition3/1
  Add1/1 -> Delay/1, vxy_est/1, Scope/1, Add/1
  Add/1 -> Rate Transition1/1
  Memory/1 -> Add1/3
  Rate Transition1/1 -> Kalman Filter/1
  Rate Transition2/1 -> Scope7/1, Kalman Filter/2
  Logical Operator/1 -> GPSv_enable/1, Rate Transition2/1, Product/2
  Product/1 -> Memory/1
  Selector/1 -> Detect Change/1
  vxy_GPS/1 -> Selector/1, Add/2, Scope/2
  Kalman Filter/1 -> Product/1
  Gain/1 -> Add1/1
  axy/1 -> Gain/1
  Delay/1 -> Add1/2

== system ZF02HD250606_23a/NavigationModel/GPSNav/1/Translation_estimate/V_Horizontal_estimation1 ==
  note: 0530改：
      | 加入GPStype限制
  An : Inport
  vn_gps : Inport  Port=2
  ve_gps : Inport  Port=3
  fixtype_gps : Inport  Port=4
  QGC_init : Inport  Port=5
  Add : Sum  Inputs=+-
  Compare To Constant : simulink/Logic and Bit Operations/Compare To Constant  relop=>=  const=3  OutDataTypeStr=boolean
  Delay : Delay  DelayLength=1
  Detect Change : simulink/Logic and Bit Operations/Detect Change  vinit=0  OutDataTypeStr=boolean
  Integrator_V_Horizontal : Subsystem
  Logical Operator : Logic  AllPortsSameDT=off  OutDataTypeStr=boolean
  Mux : Mux  Inputs=2
  Rxy_kalman filter1 : Subsystem  mask{F=diag([-0.1,-0.1,-0.002,-0.002]), H=[1,0,-1,0;0,1,0,-1], Q=diag([1,1,0.1,0.1]), R=diag([0.001,0.001]), P0=diag([0.8,0.8,0.2,0.2])}
      mask prompts: F "状态转移矩阵：F"; H "观测转移矩阵：H"; Q "预测噪声协方差矩阵：Q"; R "量测噪声协方差矩阵：R"; P0 "初始协方差矩阵：P0"
      mask DialogControl DescTextVar Prompt: Kalman Filter
  Scope : Scope  NumInputPorts=2
  Scope1 : Scope
  Selector : Selector  InputPortWidth=4  IndexOptions=Index vector (dialog)  Indices=[1 2]  OutputSizes=1
  vxy_estimout : Outport
  GPS_v_enable : Outport  Port=2
  wires:
  QGC_init/1 -> Integrator_V_Horizontal/3(QGC_init)
  Delay/1 -> Selector/1, Rxy_kalman filter1/1(X)
  Selector/1 -> Integrator_V_Horizontal/2(dv)
  vn_gps/1 -> Integrator_V_Horizontal/4(vn_gps), Mux/1, Detect Change/1
  Mux/1 -> Scope/2, Add/2
  ve_gps/1 -> Integrator_V_Horizontal/5(ve_gps), Mux/2
  Rxy_kalman filter1/1(XOut) -> Delay/1
  Integrator_V_Horizontal/1(V_n&e) -> Add/1, vxy_estimout/1, Scope/1
  Add/1 -> Rxy_kalman filter1/2(Z)
  An/1 -> Integrator_V_Horizontal/1(An)
  fixtype_gps/1 -> Compare To Constant/1
  Detect Change/1 -> Logical Operator/1
  Compare To Constant/1 -> Logical Operator/2, Scope1/1, GPS_v_enable/1, Rxy_kalman filter1/3(Enable), Integrator_V_Horizontal/6(GPSenable)

== system ZF02HD250606_23a/NavigationModel/GPSNav/1/Translation_estimate/translate to N ==
  Cbn : Inport
  accl_ned : Inport  Port=2
  Product : Product  Multiplication=Matrix(*)
  Selector : Selector  InputPortWidth=3  IndexOptions=Index vector (dialog)  Indices=[1 2]  OutputSizes=1
  accel_Horizontal_predict : Outport
  wires:
  Selector/1 -> accel_Horizontal_predict/1
  Product/1 -> Selector/1
  Cbn/1 -> Product/1
  accl_ned/1 -> Product/2

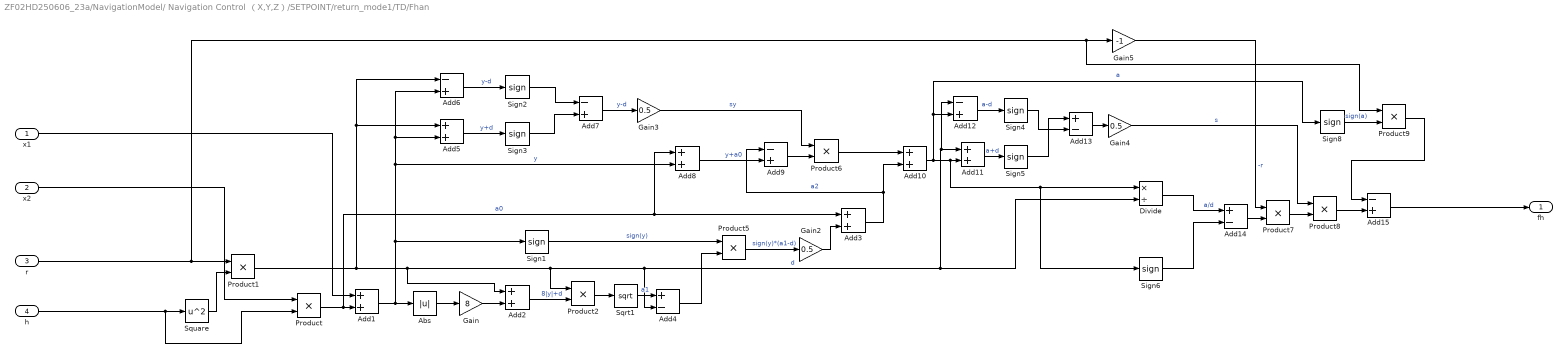
== system ZF02HD250606_23a/NavigationModel/ Navigation Control （X,Y,Z）/SETPOINT/return_mode1/TD/Fhan ==
  x1 : Inport
  x2 : Inport  Port=2
  r : Inport  Port=3
  h : Inport  Port=4
  Abs : Abs  SaturateOnIntegerOverflow=off
  Add{1..3,5,8,10..11} (7 alike) : Sum
  Add{6..7,9,12,15} (5 alike) : Sum  Inputs=-+
  Add13 : Sum  Inputs=+-
  Add14 : Sum  Inputs=+-
  Add4 : Sum  Inputs=+-
  Divide : Product  Inputs=*/
  Gain : Gain  Gain=8
  Gain2 : Gain  Gain=0.5
  Gain3 : Gain  Gain=0.5
  Gain4 : Gain  Gain=0.5
  Gain5 : Gain  Gain=-1
  Product{,1..2,5..9} (8 alike) : Product
  Sign{1..6,8} (7 alike) : Signum
  Sqrt1 : Sqrt
  Square : Math  Operator=square  SignedPower=on
  fh : Outport
  wires:
  Add1/1 -> Add8/2, Add6/2, Add5/2, Sign1/1, Abs/1  "y"
  Product1/1 -> Add6/1, Add5/1, Divide/2, Add12/1, Add11/1, Add4/2, Product2/1, Add2/1  "d"
  Add5/1 -> Sign3/1  "y+d"
  Sign4/1 -> Add13/2
  Add9/1 -> Product6/2
  Product5/1 -> Gain2/1  "sign(y)*(a1-d)"
  Gain3/1 -> Product6/1  "sy"
  Product/1 -> Add8/1, Add3/1, Add1/2  "a0"
  Product6/1 -> Add10/1
  Add7/1 -> Gain3/1  "y-d"
  Sign8/1 -> Product9/2  "sign(a)"
  Sign3/1 -> Add7/2
  Add2/1 -> Product2/2  "8|y|+d"
  r/1 -> Product9/1, Gain5/1, Product1/1
  Add10/1 -> Sign6/1, Divide/1, Add11/2, Add12/2, Sign8/1  "a"
  Product2/1 -> Sqrt1/1
  Sign5/1 -> Add13/1
  Abs/1 -> Gain/1
  Divide/1 -> Add14/1  "a/d"
  Gain2/1 -> Add3/2
  Gain/1 -> Add2/2
  Add13/1 -> Gain4/1
  Add14/1 -> Product7/2
  Add3/1 -> Add10/2, Add9/1  "a2"
  Add12/1 -> Sign4/1  "a-d"
  Gain4/1 -> Product8/1  "s"
  Product8/1 -> Add15/2
  h/1 -> Product/2, Square/1
  Square/1 -> Product1/2
  Add8/1 -> Add9/2  "y+a0"
  Sign6/1 -> Add14/2
  Add11/1 -> Sign5/1  "a+d"
  Sign2/1 -> Add7/1
  Sqrt1/1 -> Add4/1  "a1"
  Product9/1 -> Add15/1
  Add4/1 -> Product5/2
  Add6/1 -> Sign2/1  "y-d"
  Sign1/1 -> Product5/1  "sign(y)"
  Product7/1 -> Product8/2
  Gain5/1 -> Product7/1  "-r"
  x1/1 -> Add1/1
  x2/1 -> Product/1
  Add15/1 -> fh/1

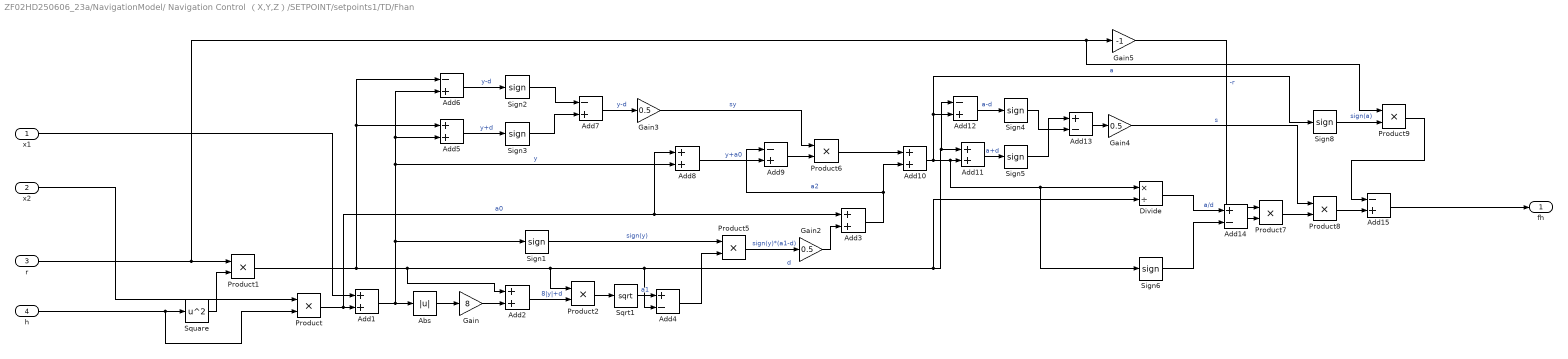
== system ZF02HD250606_23a/NavigationModel/ Navigation Control （X,Y,Z）/SETPOINT/setpoints1/TD/Fhan ==
  x1 : Inport
  x2 : Inport  Port=2
  r : Inport  Port=3
  h : Inport  Port=4
  Abs : Abs  SaturateOnIntegerOverflow=off
  Add{1..3,5,8,10..11} (7 alike) : Sum
  Add{6..7,9,12,15} (5 alike) : Sum  Inputs=-+
  Add13 : Sum  Inputs=+-
  Add14 : Sum  Inputs=+-
  Add4 : Sum  Inputs=+-
  Divide : Product  Inputs=*/
  Gain : Gain  Gain=8
  Gain2 : Gain  Gain=0.5
  Gain3 : Gain  Gain=0.5
  Gain4 : Gain  Gain=0.5
  Gain5 : Gain  Gain=-1
  Product{,1..2,5..9} (8 alike) : Product
  Sign{1..6,8} (7 alike) : Signum
  Sqrt1 : Sqrt
  Square : Math  Operator=square  SignedPower=on
  fh : Outport
  wires:
  Add1/1 -> Add8/2, Add6/2, Add5/2, Sign1/1, Abs/1  "y"
  Product1/1 -> Add6/1, Add5/1, Divide/2, Add12/1, Add11/1, Add4/2, Product2/1, Add2/1  "d"
  Add5/1 -> Sign3/1  "y+d"
  Sign4/1 -> Add13/2
  Add9/1 -> Product6/2
  Product5/1 -> Gain2/1  "sign(y)*(a1-d)"
  Gain3/1 -> Product6/1  "sy"
  Product/1 -> Add8/1, Add3/1, Add1/2  "a0"
  Product6/1 -> Add10/1
  Add7/1 -> Gain3/1  "y-d"
  Sign8/1 -> Product9/2  "sign(a)"
  Sign3/1 -> Add7/2
  Add2/1 -> Product2/2  "8|y|+d"
  r/1 -> Product9/1, Gain5/1, Product1/1
  Add10/1 -> Sign6/1, Divide/1, Add11/2, Add12/2, Sign8/1  "a"
  Product2/1 -> Sqrt1/1
  Sign5/1 -> Add13/1
  Abs/1 -> Gain/1
  Divide/1 -> Add14/1  "a/d"
  Gain2/1 -> Add3/2
  Gain/1 -> Add2/2
  Add13/1 -> Gain4/1
  Add14/1 -> Product7/2
  Add3/1 -> Add10/2, Add9/1  "a2"
  Add12/1 -> Sign4/1  "a-d"
  Gain4/1 -> Product8/1  "s"
  Product8/1 -> Add15/2
  h/1 -> Product/2, Square/1
  Square/1 -> Product1/2
  Add8/1 -> Add9/2  "y+a0"
  Sign6/1 -> Add14/2
  Add11/1 -> Sign5/1  "a+d"
  Sign2/1 -> Add7/1
  Sqrt1/1 -> Add4/1  "a1"
  Product9/1 -> Add15/1
  Add4/1 -> Product5/2
  Add6/1 -> Sign2/1  "y-d"
  Sign1/1 -> Product5/1  "sign(y)"
  Product7/1 -> Product8/2
  Gain5/1 -> Product7/1  "-r"
  x1/1 -> Add1/1
  x2/1 -> Product/1
  Add15/1 -> fh/1

== system ZF02HD250606_23a/NavigationModel/GPSNav/1/Translation_estimate/V_Horizontal_estimation1/Integrator_V_Horizontal ==
  An : Inport
  dv : Inport  Port=2
  QGC_init : Inport  Port=3
  vn_gps : Inport  Port=4
  ve_gps : Inport  Port=5
  GPSenable : Inport  Port=6
  Delay : Delay  DelayLength=1  InitialConditionSource=Input port  ExternalReset=Rising
      settings: InputPortMap=u0,r5,p4
  Gain : Gain  Gain=0.8
  Gain2 : Gain  Gain=dt  SaturateOnIntegerOverflow=on  OutDataTypeStr=Inherit: Same as input  ParamDataTypeStr=Inherit: Same as input
  Mux : Mux  Inputs=2
  Product : Product
  Scope : Scope
  Sum : Sum  Inputs=|++-
  V_n&e : Outport
  wires:
  GPSenable/1 -> Product/2
  dv/1 -> Product/1
  An/1 -> Gain2/1
  Gain2/1 -> Sum/1
  Sum/1 -> V_n&e/1, Delay/1
  QGC_init/1 -> Delay/2
  vn_gps/1 -> Mux/1
  ve_gps/1 -> Mux/2
  Mux/1 -> Delay/3
  Delay/1 -> Sum/2
  Product/1 -> Gain/1
  Gain/1 -> Scope/1, Sum/3

== system ZF02HD250606_23a/NavigationModel/GPSNav/1/Translation_estimate/V_Horizontal_estimation1/Rxy_kalman filter1 ==
  X : Inport
  Z : Inport  Port=2
  Enable : Inport  Port=3
  Constant : Constant  Value=F  OutDataTypeStr=single
  Constant1 : Constant  Value=Q  OutDataTypeStr=single
  Constant2 : Constant  Value=R  OutDataTypeStr=single
  Constant3 : Constant  Value=P0  OutDataTypeStr=single
  Constant4 : Constant  Value=H  OutDataTypeStr=single
  Vxy kalman filter : Subsystem  TreatAsAtomicUnit=on
  XOut : Outport
  wires:
  Enable/1 -> Vxy kalman filter/9(Enable)
  Vxy kalman filter/1(XOut) -> XOut/1
  Constant1/1 -> Vxy kalman filter/5(Q)
  Constant4/1 -> Vxy kalman filter/4(H)
  Constant2/1 -> Vxy kalman filter/6(R)
  Constant3/1 -> Vxy kalman filter/8(P0)
  Z/1 -> Vxy kalman filter/1(Z)
  Constant/1 -> Vxy kalman filter/3(G), Vxy kalman filter/2(F)
  X/1 -> Vxy kalman filter/7(X)

== system ZF02HD250606_23a/NavigationModel/GPSNav/1/Translation_estimate/V_Horizontal_estimation1/Rxy_kalman filter1/Vxy kalman filter ==
  Z : Inport
  F : Inport  Port=2
  G : Inport  Port=3
  H : Inport  Port=4
  Q : Inport  Port=5
  R : Inport  Port=6
  X : Inport  Port=7
  P0 : Inport  Port=8
  Enable : Inport  Port=9
  Add1 : Sum
  Delay : Delay  DelayLength=1  InitialConditionSource=Input port
      settings: InputPortMap=u0,p4
  Gain4 : Gain  Gain=0.5
  Math Function : Math  Operator=transpose  SignedPower=on
  kalman : Subsystem
  XOut : Outport
  wires:
  P0/1 -> Delay/2
  Gain4/1 -> Delay/1
  Delay/1 -> kalman/7(P)
  Add1/1 -> Gain4/1
  Math Function/1 -> Add1/2
  Z/1 -> kalman/1(Z)
  F/1 -> kalman/2(F)
  G/1 -> kalman/3(G)
  H/1 -> kalman/4(H)
  Q/1 -> kalman/5(Q)
  R/1 -> kalman/6(R)
  X/1 -> kalman/8(X)
  kalman/1(POut) -> Math Function/1, Add1/1
  kalman/2(XOut) -> XOut/1
  Enable/1 -> kalman/9(Enable)

== system ZF02HD250606_23a/NavigationModel/GPSNav/1/Translation_estimate/V_Horizontal_estimation1/Rxy_kalman filter1/Vxy kalman filter/kalman ==
  note: Xk/k-1=FXk-1
      | Xk=Xk/k-1+K(Z-h(Xk/k-1))
      | K=Pk/k-1H(HPk/k-1H+Rk)-1
      | Pk/k-1=FPk-1F+GQG
      | Pk=(I-KH)Pk/k-1
  Z : Inport
  F : Inport  Port=2
  G : Inport  Port=3
  H : Inport  Port=4
  Q : Inport  Port=5
  R : Inport  Port=6
  P : Inport  Port=7
  X : Inport  Port=8
  Enable : Inport  Port=9
  Scope : Scope  NumInputPorts=2
  Subsystem : Subsystem
  Subsystem1 : Subsystem
  POut : Outport
  XOut : Outport  Port=2
  wires:
  X/1 -> [X]
  P/1 -> [P]
  Q/1 -> [Q]
  G/1 -> [G]
  F/1 -> [F]
  Z/1 -> [Z]
  [F] -> Subsystem/1(F)
  [G] -> Subsystem/2(G)
  [Q] -> Subsystem/3(Q)
  [X] -> Subsystem/4(X)
  [P] -> Subsystem/5(P)
  Subsystem/1(Xk_k_1) -> [Xk_k_1]
  Subsystem/2(Pk_k_1) -> [Pk_k_1]
  H/1 -> Subsystem1/3(H)
  R/1 -> Subsystem1/4(R)
  Subsystem1/1(POut) -> POut/1
  Subsystem1/2(XOut) -> XOut/1, Scope/2
  [Xk_k_1] -> Subsystem1/1(Xkk)
  [Pk_k_1] -> Subsystem1/2(Pkk)
  Enable/1 -> Subsystem1/Enable, Scope/1
  [Z] -> Subsystem1/5(Z)

== system ZF02HD250606_23a/NavigationModel/GPSNav/1/Translation_estimate/V_Horizontal_estimation1/Rxy_kalman filter1/Vxy kalman filter/kalman/Subsystem ==
  F : Inport
  G : Inport  Port=2
  Q : Inport  Port=3
  X : Inport  Port=4
  P : Inport  Port=5
  Add : Sum
  Math Function3 : Math  Operator=transpose  SignedPower=on
  Math Function4 : Math  Operator=transpose  SignedPower=on
  MatrixMultiply : Product  Multiplication=Matrix(*)
  MatrixMultiply1 : Product  Inputs=3  Multiplication=Matrix(*)
  MatrixMultiply8 : Product  Inputs=3  Multiplication=Matrix(*)
  Xk_k_1 : Outport
  Pk_k_1 : Outport  Port=2
  wires:
  Math Function4/1 -> MatrixMultiply8/3
  [Q] -> MatrixMultiply8/2
  MatrixMultiply/1 -> [Xk_k_1]
  MatrixMultiply1/1 -> Add/1
  [F] -> Math Function3/1
  Math Function3/1 -> MatrixMultiply1/3
  [P] -> MatrixMultiply1/2
  [F] -> MatrixMultiply1/1
  Add/1 -> [Pk_k_1]
  [G] -> MatrixMultiply8/1
  MatrixMultiply8/1 -> Add/2
  [X] -> MatrixMultiply/2
  [G] -> Math Function4/1
  [F] -> MatrixMultiply/1
  F/1 -> [F]
  G/1 -> [G]
  Q/1 -> [Q]
  X/1 -> [X]
  P/1 -> [P]
  [Xk_k_1] -> Xk_k_1/1
  [Pk_k_1] -> Pk_k_1/1

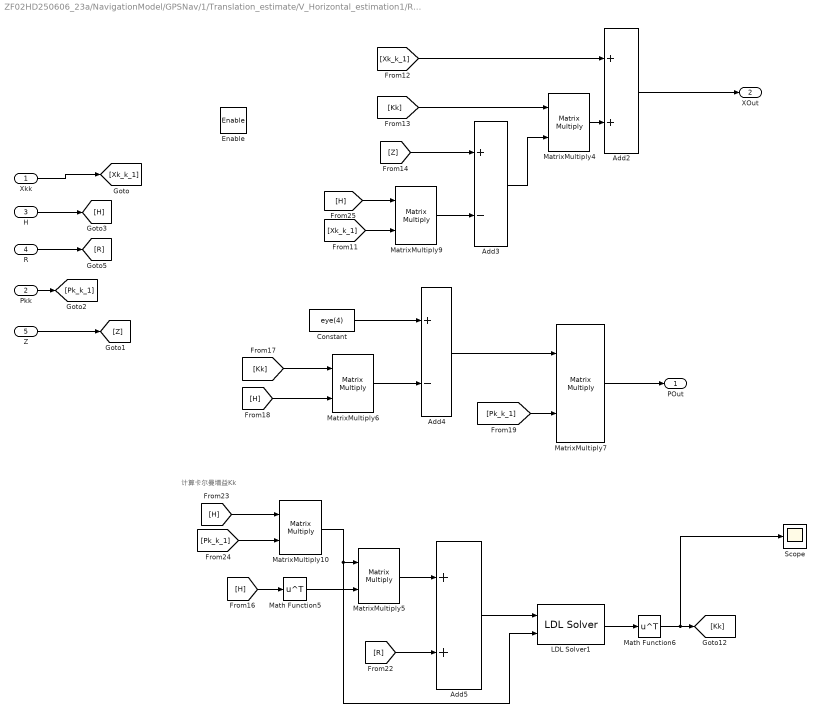
== system ZF02HD250606_23a/NavigationModel/GPSNav/1/Translation_estimate/V_Horizontal_estimation1/Rxy_kalman filter1/Vxy kalman filter/kalman/Subsystem1 ==
  note: 计算卡尔曼增益Kk
  Xkk : Inport
  Pkk : Inport  Port=2
  H : Inport  Port=3
  R : Inport  Port=4
  Z : Inport  Port=5
  Enable : EnablePort
  Add2 : Sum
  Add3 : Sum  Inputs=+-
  Add4 : Sum  Inputs=+-
  Add5 : Sum
  Constant : Constant  Value=eye(4)  OutDataTypeStr=single
  LDL Solver1 : dspsolvers/LDL Solver  errmode=Warning
      settings: RTWMemSecFuncInitTerm=Default  RTWMemSecFuncExecute=Default  RTWMemSecDataConstants=Default  RTWMemSecDataInternal=Default  RTWMemSecDataParameters=Default
  Math Function5 : Math  Operator=transpose  SignedPower=on
  Math Function6 : Math  Operator=transpose  SignedPower=on
  MatrixMultiply{4..7,9..10} (6 alike) : Product  Multiplication=Matrix(*)
  Scope : Scope
  POut : Outport
  XOut : Outport  Port=2
  wires:
  MatrixMultiply9/1 -> Add3/2
  MatrixMultiply7/1 -> POut/1
  [H] -> MatrixMultiply10/1
  Add3/1 -> MatrixMultiply4/2
  Math Function5/1 -> MatrixMultiply5/2
  Math Function6/1 -> Scope/1, [Kk]
  Add4/1 -> MatrixMultiply7/1
  MatrixMultiply4/1 -> Add2/2
  [Kk] -> MatrixMultiply4/1
  [Z] -> Add3/1
  MatrixMultiply10/1 -> MatrixMultiply5/1, LDL Solver1/2
  MatrixMultiply5/1 -> Add5/1
  LDL Solver1/1 -> Math Function6/1
  [H] -> Math Function5/1
  [Pk_k_1] -> MatrixMultiply10/2
  [R] -> Add5/2
  Constant/1 -> Add4/1
  [Kk] -> MatrixMultiply6/1
  [Xk_k_1] -> Add2/1
  [H] -> MatrixMultiply6/2
  [H] -> MatrixMultiply9/1
  [Xk_k_1] -> MatrixMultiply9/2
  [Pk_k_1] -> MatrixMultiply7/2
  R/1 -> [R]
  Add5/1 -> LDL Solver1/1
  MatrixMultiply6/1 -> Add4/2
  H/1 -> [H]
  Add2/1 -> XOut/1
  Xkk/1 -> [Xk_k_1]
  Z/1 -> [Z]
  Pkk/1 -> [Pk_k_1]

== matlab function ZF02HD250606_23a/RCScheduleModel/Yaw_control/MATLAB Function2 ==
  data: u input; des_wz output; Yaw input; Yaw_dei input
function des_wz = fcn(u, Yaw, Yaw_dei)
% ctrlChCmdAPI[3]=[-7875,8897]

%偏航指令： [-20,20]
des_psi = u/440 +Yaw_dei;  % 为了使得量级对应， [-7875,8897]/[-20,20]约等于440
%des_psi = 0;
erro_psi = des_psi-Yaw*57.3;
P = 200;   %将正负20°的航向角误差转化为期望的偏航角速率
k= 0.42;  % V5.05.241021将K值由1更改为0.5、0.4、0.1、0.27、0.35、0.42
des_wz = P*k*erro_psi;

end

== matlab function ZF02HD250606_23a/RCScheduleModel/MATLAB Function ==
  data: roll0 input; pitch0 input; u input; y output; data input
function y = fcn(roll0,pitch0,u, data)
y = zeros(4,1);
y(1) = data(1)+roll0 ;
y(2) =  data(2)+pitch0;
y(3) = u(3);
y(4) = u(4)+data(3);
end

== stateflow chart ZF02HD250606_23a/NavigationModel/ Navigation Control （X,Y,Z）/SETPOINT/setpoints1/Chart ==
  state Line
    en, du: flag_setpoint = 0;
  state Next
    en, du: flag_setpoint = 1;
  (default) -> Line
  Next -> Line : [dist < 1 ]
  Line -> Next : [dist > 0]
  data: dist input; flag_setpoint output
